simulink model "modelo_3_naolinear"  (R2026a)
settings: Solver=ode45  StopTime=8

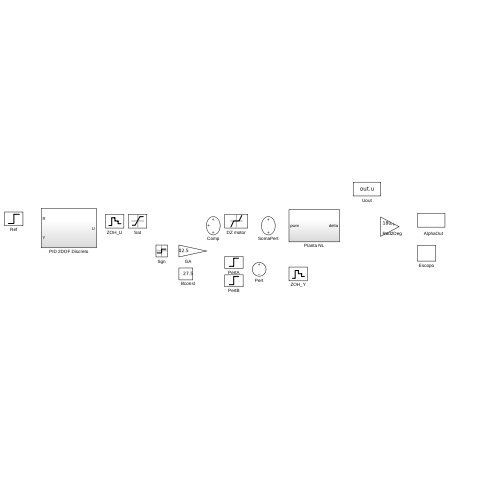
[thumbnail: Simulink's stored preview of the top-level diagram]
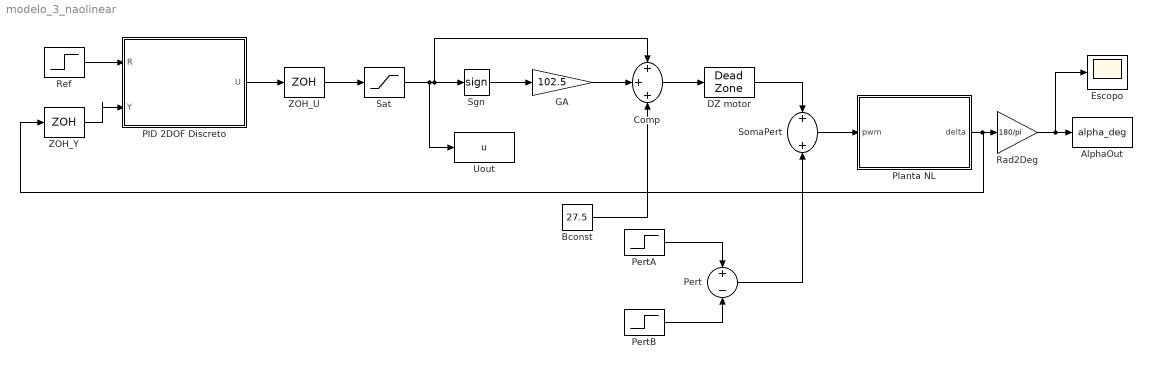
== system modelo_3_naolinear ==
  AlphaOut : ToWorkspace  VariableName=alpha_deg  SaveFormat=Timeseries  SampleTime=-1
  Bconst : Constant  Value=27.5
  Comp : Sum  Inputs=+++
  DZ motor : DeadZone  LowerValue=-75  UpperValue=130
  Escopo : Scope
  GA : Gain  Gain=102.5
  PID 2DOF Discreto : Subsystem
  Pert : Sum  Inputs=+-
  PertA : Step  Time=2  FinalValue=60  SampleTime=0
  PertB : Step  Time=2.3  FinalValue=60  SampleTime=0
  Planta NL : Subsystem
  Rad2Deg : Gain  Gain=180/pi
  Ref : Step  Time=0  FinalValue=0  SampleTime=0
  Sat : Saturate  UpperLimit=255  LowerLimit=-255
  Sgn : Signum
  SomaPert : Sum
  Uout : ToWorkspace  VariableName=u  SaveFormat=Timeseries  SampleTime=-1
  ZOH_U : ZeroOrderHold  SampleTime=0.02
  ZOH_Y : ZeroOrderHold  SampleTime=0.02
  wires:
  Planta NL/1(delta) -> Rad2Deg/1, ZOH_Y/1
  Ref/1 -> PID 2DOF Discreto/1(R)
  ZOH_Y/1 -> PID 2DOF Discreto/2(Y)
  DZ motor/1 -> SomaPert/1
  Pert/1 -> SomaPert/2
  PID 2DOF Discreto/1(U) -> ZOH_U/1
  ZOH_U/1 -> Sat/1
  Rad2Deg/1 -> Escopo/1, AlphaOut/1
  SomaPert/1 -> Planta NL/1(pwm)
  PertB/1 -> Pert/2
  GA/1 -> Comp/2
  Sat/1 -> Sgn/1, Comp/1, Uout/1
  Sgn/1 -> GA/1
  Bconst/1 -> Comp/3
  PertA/1 -> Pert/1
  Comp/1 -> DZ motor/1

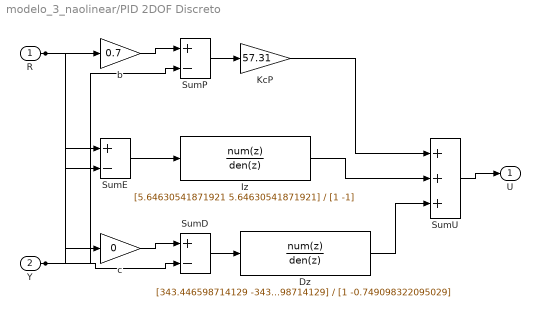
== system modelo_3_naolinear/PID 2DOF Discreto ==
  R : Inport
  Y : Inport  Port=2
  Dz : DiscreteTransferFcn  Numerator=[343.446598714129 -343.446598714129]  Denominator=[1 -0.749098322095029]  SampleTime=0.02
  Iz : DiscreteTransferFcn  Numerator=[5.64630541871921 5.64630541871921]  Denominator=[1 -1]  SampleTime=0.02
  KcP : Gain  Gain=57.31
  SumD : Sum  Inputs=+-
  SumE : Sum  Inputs=+-
  SumP : Sum  Inputs=+-
  SumU : Sum  Inputs=+++
  b : Gain  Gain=0.7
  c : Gain  Gain=0
  U : Outport
  wires:
  R/1 -> b/1, SumE/1, c/1
  b/1 -> SumP/1
  Y/1 -> SumP/2, SumE/2, SumD/2
  SumP/1 -> KcP/1
  SumE/1 -> Iz/1
  c/1 -> SumD/1
  SumD/1 -> Dz/1
  KcP/1 -> SumU/1
  Iz/1 -> SumU/2
  Dz/1 -> SumU/3
  SumU/1 -> U/1

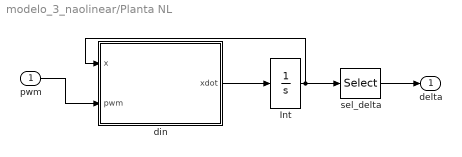
== system modelo_3_naolinear/Planta NL ==
  pwm : Inport
  Int : Integrator  InitialCondition=[0;0;0;0]
  din : MATLAB Function  TreatAsAtomicUnit=on
  sel_delta : Selector  InputPortWidth=4  IndexOptions=Index vector (dialog)  Indices=2  OutputSizes=1
  delta : Outport
  wires:
  pwm/1 -> din/2(pwm)
  Int/1 -> din/1(x), sel_delta/1
  din/1(xdot) -> Int/1
  sel_delta/1 -> delta/1

== matlab function modelo_3_naolinear/Planta NL/din ==
  data: x input; xdot output; pwm input
function xdot = din(x, pwm)
%#codegen
k_tau = 0.00050868; Ib = 0.0015; mp = 0.045; Lb = 0.12; J = 0.00051271;
lp = 0.08; b_th = 1e-05; b_al = 0.00057586; g = 9.81;
th_d = x(3); d = x(2); d_d = x(4);
tau  = k_tau*pwm;
M11 = Ib + mp*Lb^2 + J*sin(d)^2;
M12 = -mp*Lb*lp*cos(d);
M22 = J;
C1  = J*sin(2*d)*th_d*d_d + mp*Lb*lp*sin(d)*d_d^2;
C2  = -0.5*J*sin(2*d)*th_d^2;
r1  = tau - C1 - b_th*th_d;
r2  =     - C2 - b_al*d_d - mp*g*lp*sin(d);
det = M11*M22 - M12^2;
th_dd = ( M22*r1 - M12*r2)/det;
d_dd  = (-M12*r1 + M11*r2)/det;
xdot  = [th_d; d_d; th_dd; d_dd];
